simulink model "stewart_platform_model"  (R2025b)
settings: Solver=ode45  StartTime=0.0  StopTime=0.1  FixedStep=1e-4  MaxStep=0.2  RelTol=1e-4  AbsTol=1e-4
values from neighbouring files (symbols this model uses):
  ground = initializeGround('type', 'none')    [active_damping_dvf.m]    (also in active_damping_iff.m; active_damping_inertial.m; cubic_conf_coupling_cartesianl.m; cubic_conf_coupling_strutsl.m)
  payload = initializePayload('type', 'none')    [active_damping_dvf.m]    (also in active_damping_iff.m; active_damping_inertial.m; cubic_conf_coupling_cartesianl.m; cubic_conf_coupling_strutsl.m)
  s = zpk('s')    [active_damping_dvf.m]    (also in active_damping_iff.m; active_damping_inertial.m; cubic_conf_above_platforml.m; cubic_conf_coupling_cartesianl.m)
undefined symbols (not defined in the file or in its folder): X, Y, Z
libraries: sm_lib x29, nesl_utility x27, cstblocks x10
(part 2 of 2)

== system stewart_platform_model/Payload/Cartesian ==
  Cartesian Joint : sm_lib/Joints/Cartesian Joint  JointMode=Normal  CompositeWrenchDir=FollowerOnBase  CompositeWrenchFrame=BaseFrame  SenseConstraintForce=off  SenseConstraintTorque=off  SenseTotalForce=off  SenseTotalTorque=off  PxPositionTargetSpecify=off  PxPositionTargetPriority=High  PxPositionTargetValue=0  PxPositionTargetValueUnits=m  PxVelocityTargetSpecify=off  PxVelocityTargetPriority=High  PxVelocityTargetValue=0  PxVelocityTargetValueUnits=m/s  PxEquilibriumPosition=0  PxEquilibriumPositionUnits=m  PxSpringStiffness=payload.K(1)  PxSpringStiffnessUnits=N/m  PxDampingCoefficient=payload.C(1)  PxDampingCoefficientUnits=N/(m/s)  PxLowerLimitSpecify=off  PxLowerLimitBound=-1  PxLowerLimitBoundUnits=m  PxLowerLimitStiffness=1e6  PxLowerLimitStiffnessUnits=N/m  PxLowerLimitDamping=1e3  PxLowerLimitDampingUnits=N/(m/s)  PxLowerLimitTransitionRegionWidth=1e-4  PxLowerLimitTransitionRegionWidthUnits=m  PxUpperLimitSpecify=off  PxUpperLimitBound=1  PxUpperLimitBoundUnits=m  PxUpperLimitStiffness=1e6  PxUpperLimitStiffnessUnits=N/m  PxUpperLimitDamping=1e3  PxUpperLimitDampingUnits=N/(m/s)  PxUpperLimitTransitionRegionWidth=1e-4  PxUpperLimitTransitionRegionWidthUnits=m  PxTorqueActuationMode=NoTorque  PxMotionActuationMode=ComputedMotion  PxSensePosition=off  PxSenseVelocity=off  PxSenseAcceleration=off  PxSenseTorqueForce=off  PxSenseLowerLimitTorqueForce=off  PxSenseUpperLimitTorqueForce=off  PyPositionTargetSpecify=off  PyPositionTargetPriority=High  PyPositionTargetValue=0  PyPositionTargetValueUnits=m  PyVelocityTargetSpecify=off  PyVelocityTargetPriority=High  PyVelocityTargetValue=0  PyVelocityTargetValueUnits=m/s  PyEquilibriumPosition=0  PyEquilibriumPositionUnits=m  PySpringStiffness=payload.K(2)  PySpringStiffnessUnits=N/m  PyDampingCoefficient=payload.C(2)  PyDampingCoefficientUnits=N/(m/s)  PyLowerLimitSpecify=off  PyLowerLimitBound=-1  PyLowerLimitBoundUnits=m  PyLowerLimitStiffness=1e6  PyLowerLimitStiffnessUnits=N/m  PyLowerLimitDamping=1e3  PyLowerLimitDampingUnits=N/(m/s)  PyLowerLimitTransitionRegionWidth=1e-4  PyLowerLimitTransitionRegionWidthUnits=m  PyUpperLimitSpecify=off  PyUpperLimitBound=1  PyUpperLimitBoundUnits=m  PyUpperLimitStiffness=1e6  PyUpperLimitStiffnessUnits=N/m  PyUpperLimitDamping=1e3  PyUpperLimitDampingUnits=N/(m/s)  PyUpperLimitTransitionRegionWidth=1e-4  PyUpperLimitTransitionRegionWidthUnits=m  PyTorqueActuationMode=NoTorque  PyMotionActuationMode=ComputedMotion  PySensePosition=off  PySenseVelocity=off  PySenseAcceleration=off  PySenseTorqueForce=off  PySenseLowerLimitTorqueForce=off  PySenseUpperLimitTorqueForce=off  PzPositionTargetSpecify=off  PzPositionTargetPriority=High  PzPositionTargetValue=0  PzPositionTargetValueUnits=m  PzVelocityTargetSpecify=off  PzVelocityTargetPriority=High  PzVelocityTargetValue=0  PzVelocityTargetValueUnits=m/s  PzEquilibriumPosition=0  PzEquilibriumPositionUnits=m  PzSpringStiffness=payload.K(3)  PzSpringStiffnessUnits=N/m  PzDampingCoefficient=payload.C(3)  PzDampingCoefficientUnits=N/(m/s)  PzLowerLimitSpecify=off  PzLowerLimitBound=-1  PzLowerLimitBoundUnits=m  PzLowerLimitStiffness=1e6  PzLowerLimitStiffnessUnits=N/m  PzLowerLimitDamping=1e3  PzLowerLimitDampingUnits=N/(m/s)  PzLowerLimitTransitionRegionWidth=1e-4  PzLowerLimitTransitionRegionWidthUnits=m  PzUpperLimitSpecify=off  PzUpperLimitBound=1  PzUpperLimitBoundUnits=m  PzUpperLimitStiffness=1e6  PzUpperLimitStiffnessUnits=N/m  PzUpperLimitDamping=1e3  PzUpperLimitDampingUnits=N/(m/s)  PzUpperLimitTransitionRegionWidth=1e-4  PzUpperLimitTransitionRegionWidthUnits=m  PzTorqueActuationMode=NoTorque  PzMotionActuationMode=ComputedMotion  PzSensePosition=off  PzSenseVelocity=off  PzSenseAcceleration=off  PzSenseTorqueForce=off  PzSenseLowerLimitTorqueForce=off  PzSenseUpperLimitTorqueForce=off
  Cylindrical Solid : sm_lib/Body Elements/Cylindrical Solid  CylinderRadius=0.1  CylinderRadiusUnits=m  CylinderLength=2*payload.h  CylinderLengthUnits=m  ExportEntireGeometry=off  InertiaType=Custom  BasedOnType=Mass  Density=1000  DensityUnits=kg/m^3  Mass=payload.m  MassUnits=kg  CenterOfMass=[0 0 payload.h]  CenterOfMassUnits=m  MomentsOfInertia=diag(payload.I)  MomentsOfInertiaUnits=kg*m^2  ProductsOfInertia=[payload.I(2,3) payload.I(1,3) payload.I(1,2)]  ProductsOfInertiaUnits=kg*m^2  GraphicType=FromGeometry  MarkerShape=Sphere  MarkerSize=10  GraphicVisPropType=SimpleVisualProperties  GraphicDiffuseColor=[0.5 0.5 0.5]  GraphicOpacity=1.0  GraphicSpecularColor=[0.5 0.5 0.5 1.0]  GraphicAmbientColor=[0.15 0.15 0.15 1.0]  GraphicEmissiveColor=[0.0 0.0 0.0 1.0]  GraphicShininess=75  DoExposeReferenceFrame=on  SerializedFrames=<Frames/>
  Rigid Transform : sm_lib/Frames and Transforms/Rigid Transform  RotationMethod=None  FollAlignAxisA=+X  BaseAlignAxisA=+Y  FollAlignAxisB=+Y  BaseAlignAxisB=+Z  RotationStandardAxis=+Z  RotationAngle=0.0  RotationAngleUnits=deg  RotationArbitraryAxis=[0 0 1]  RotationSequenceAxes=FollowerAxes  RotationSequence=XYX  RotationSequenceAngles=[0 0 0]  RotationSequenceAnglesUnits=deg  RotationMatrix=[1 0 0; 0 1 0; 0 0 1]  Quaternion=[1 0 0 0]  TranslationMethod=StandardAxis  TranslationCartesianOffset=[0 0 0]  TranslationCartesianOffsetUnits=m  TranslationStandardAxis=+Z  TranslationStandardOffset=payload.h  TranslationStandardOffsetUnits=m  TranslationROffset=0  TranslationROffsetUnits=m  TranslationThetaOffset=0  TranslationThetaOffsetUnits=deg  TranslationZOffset=0  TranslationZOffsetUnits=m
  Rigid Transform1 : sm_lib/Frames and Transforms/Rigid Transform  RotationMethod=None  FollAlignAxisA=+X  BaseAlignAxisA=+Y  FollAlignAxisB=+Y  BaseAlignAxisB=+Z  RotationStandardAxis=+Z  RotationAngle=0.0  RotationAngleUnits=deg  RotationArbitraryAxis=[0 0 1]  RotationSequenceAxes=FollowerAxes  RotationSequence=XYX  RotationSequenceAngles=[0 0 0]  RotationSequenceAnglesUnits=deg  RotationMatrix=[1 0 0; 0 1 0; 0 0 1]  Quaternion=[1 0 0 0]  TranslationMethod=StandardAxis  TranslationCartesianOffset=[0 0 0]  TranslationCartesianOffsetUnits=m  TranslationStandardAxis=+Z  TranslationStandardOffset=payload.h  TranslationStandardOffsetUnits=m  TranslationROffset=0  TranslationROffsetUnits=m  TranslationThetaOffset=0  TranslationThetaOffsetUnits=deg  TranslationZOffset=0  TranslationZOffsetUnits=m
  Rigid Transform2 : sm_lib/Frames and Transforms/Rigid Transform  RotationMethod=None  FollAlignAxisA=+X  BaseAlignAxisA=+Y  FollAlignAxisB=+Y  BaseAlignAxisB=+Z  RotationStandardAxis=+Z  RotationAngle=0.0  RotationAngleUnits=deg  RotationArbitraryAxis=[0 0 1]  RotationSequenceAxes=FollowerAxes  RotationSequence=XYX  RotationSequenceAngles=[0 0 0]  RotationSequenceAnglesUnits=deg  RotationMatrix=[1 0 0; 0 1 0; 0 0 1]  Quaternion=[1 0 0 0]  TranslationMethod=Cartesian  TranslationCartesianOffset=stewart.platform_M.MO_B  TranslationCartesianOffsetUnits=m  TranslationStandardAxis=+Z  TranslationStandardOffset=0  TranslationStandardOffsetUnits=m  TranslationROffset=0  TranslationROffsetUnits=m  TranslationThetaOffset=0  TranslationThetaOffsetUnits=deg  TranslationZOffset=0  TranslationZOffsetUnits=m
  "{M}" : PMIOPort  Side=Left
  "{P}" : PMIOPort  Port=2  Side=Right
  connections:
  Cartesian Joint/LConn1 -- Rigid Transform/RConn1
  Rigid Transform/LConn1 -- "{M}"/RConn1
  Cartesian Joint/RConn1 -- Rigid Transform1/RConn1 -- Cylindrical Solid/RConn1
  "{P}"/RConn1 -- Rigid Transform2/RConn1
  Rigid Transform2/LConn1 -- Rigid Transform1/LConn1

== system stewart_platform_model/Payload/Flexible ==
  Bushing Joint : sm_lib/Joints/Bushing Joint  JointMode=Normal  CompositeWrenchDir=FollowerOnBase  CompositeWrenchFrame=BaseFrame  SenseConstraintForce=off  SenseConstraintTorque=off  SenseTotalForce=off  SenseTotalTorque=off  PxPositionTargetSpecify=off  PxPositionTargetPriority=High  PxPositionTargetValue=0  PxPositionTargetValueUnits=m  PxVelocityTargetSpecify=off  PxVelocityTargetPriority=High  PxVelocityTargetValue=0  PxVelocityTargetValueUnits=m/s  PxEquilibriumPosition=0  PxEquilibriumPositionUnits=m  PxSpringStiffness=payload.K(1)  PxSpringStiffnessUnits=N/m  PxDampingCoefficient=payload.C(1)  PxDampingCoefficientUnits=N/(m/s)  PxLowerLimitSpecify=off  PxLowerLimitBound=-1  PxLowerLimitBoundUnits=m  PxLowerLimitStiffness=1e6  PxLowerLimitStiffnessUnits=N/m  PxLowerLimitDamping=1e3  PxLowerLimitDampingUnits=N/(m/s)  PxLowerLimitTransitionRegionWidth=1e-4  PxLowerLimitTransitionRegionWidthUnits=m  PxUpperLimitSpecify=off  PxUpperLimitBound=1  PxUpperLimitBoundUnits=m  PxUpperLimitStiffness=1e6  PxUpperLimitStiffnessUnits=N/m  PxUpperLimitDamping=1e3  PxUpperLimitDampingUnits=N/(m/s)  PxUpperLimitTransitionRegionWidth=1e-4  PxUpperLimitTransitionRegionWidthUnits=m  PxTorqueActuationMode=NoTorque  PxMotionActuationMode=ComputedMotion  PxSensePosition=off  PxSenseVelocity=off  PxSenseAcceleration=off  PxSenseTorqueForce=off  PxSenseLowerLimitTorqueForce=off  PxSenseUpperLimitTorqueForce=off  PyPositionTargetSpecify=off  PyPositionTargetPriority=High  PyPositionTargetValue=0  PyPositionTargetValueUnits=m  PyVelocityTargetSpecify=off  PyVelocityTargetPriority=High  PyVelocityTargetValue=0  PyVelocityTargetValueUnits=m/s  PyEquilibriumPosition=0  PyEquilibriumPositionUnits=m  PySpringStiffness=payload.K(2)  PySpringStiffnessUnits=N/m  PyDampingCoefficient=payload.C(2)  PyDampingCoefficientUnits=N/(m/s)  PyLowerLimitSpecify=off  PyLowerLimitBound=-1  PyLowerLimitBoundUnits=m  PyLowerLimitStiffness=1e6  PyLowerLimitStiffnessUnits=N/m  PyLowerLimitDamping=1e3  PyLowerLimitDampingUnits=N/(m/s)  PyLowerLimitTransitionRegionWidth=1e-4  PyLowerLimitTransitionRegionWidthUnits=m  PyUpperLimitSpecify=off  PyUpperLimitBound=1  PyUpperLimitBoundUnits=m  PyUpperLimitStiffness=1e6  PyUpperLimitStiffnessUnits=N/m  PyUpperLimitDamping=1e3  PyUpperLimitDampingUnits=N/(m/s)  PyUpperLimitTransitionRegionWidth=1e-4  PyUpperLimitTransitionRegionWidthUnits=m  PyTorqueActuationMode=NoTorque  PyMotionActuationMode=ComputedMotion  PySensePosition=off  PySenseVelocity=off  PySenseAcceleration=off  PySenseTorqueForce=off  PySenseLowerLimitTorqueForce=off  PySenseUpperLimitTorqueForce=off  PzPositionTargetSpecify=off  PzPositionTargetPriority=High  PzPositionTargetValue=0  PzPositionTargetValueUnits=m  PzVelocityTargetSpecify=off  PzVelocityTargetPriority=High  PzVelocityTargetValue=0  PzVelocityTargetValueUnits=m/s  PzEquilibriumPosition=0  PzEquilibriumPositionUnits=m  PzSpringStiffness=payload.K(3)  PzSpringStiffnessUnits=N/m  PzDampingCoefficient=payload.C(3)  PzDampingCoefficientUnits=N/(m/s)  PzLowerLimitSpecify=off  PzLowerLimitBound=-1  PzLowerLimitBoundUnits=m  PzLowerLimitStiffness=1e6  PzLowerLimitStiffnessUnits=N/m  PzLowerLimitDamping=1e3  PzLowerLimitDampingUnits=N/(m/s)  PzLowerLimitTransitionRegionWidth=1e-4  PzLowerLimitTransitionRegionWidthUnits=m  PzUpperLimitSpecify=off  PzUpperLimitBound=1  PzUpperLimitBoundUnits=m  PzUpperLimitStiffness=1e6  PzUpperLimitStiffnessUnits=N/m  PzUpperLimitDamping=1e3  PzUpperLimitDampingUnits=N/(m/s)  PzUpperLimitTransitionRegionWidth=1e-4  PzUpperLimitTransitionRegionWidthUnits=m  PzTorqueActuationMode=NoTorque  PzMotionActuationMode=ComputedMotion  PzSensePosition=off  PzSenseVelocity=off  PzSenseAcceleration=off  PzSenseTorqueForce=off  PzSenseLowerLimitTorqueForce=off  PzSenseUpperLimitTorqueForce=off  RxPositionTargetSpecify=off  RxPositionTargetPriority=High  RxPositionTargetValue=0  RxPositionTargetValueUnits=deg  RxVelocityTargetSpecify=off  RxVelocityTargetPriority=High  RxVelocityTargetValue=0  RxVelocityTargetValueUnits=deg/s  RxEquilibriumPosition=0  RxEquilibriumPositionUnits=deg  RxSpringStiffness=payload.K(4)  RxSpringStiffnessUnits=N*m/rad  RxDampingCoefficient=payload.C(4)  RxDampingCoefficientUnits=N*m/(rad/s)  RxLowerLimitSpecify=off  RxLowerLimitBound=-90  RxLowerLimitBoundUnits=deg  RxLowerLimitStiffness=1e4  RxLowerLimitStiffnessUnits=N*m/deg  RxLowerLimitDamping=10  RxLowerLimitDampingUnits=N*m/(deg/s)  RxLowerLimitTransitionRegionWidth=0.1  RxLowerLimitTransitionRegionWidthUnits=deg  RxUpperLimitSpecify=off  RxUpperLimitBound=90  RxUpperLimitBoundUnits=deg  RxUpperLimitStiffness=1e4  RxUpperLimitStiffnessUnits=N*m/deg  RxUpperLimitDamping=10  RxUpperLimitDampingUnits=N*m/(deg/s)  RxUpperLimitTransitionRegionWidth=0.1  RxUpperLimitTransitionRegionWidthUnits=deg  RxTorqueActuationMode=NoTorque  RxMotionActuationMode=ComputedMotion  RxSensePosition=off  RxSenseVelocity=off  RxSenseAcceleration=off  RxSenseTorqueForce=off  RxSenseLowerLimitTorqueForce=off  RxSenseUpperLimitTorqueForce=off  RyPositionTargetSpecify=off  RyPositionTargetPriority=High  RyPositionTargetValue=0  RyPositionTargetValueUnits=deg  RyVelocityTargetSpecify=off  RyVelocityTargetPriority=High  RyVelocityTargetValue=0  RyVelocityTargetValueUnits=deg/s  RyEquilibriumPosition=0  RyEquilibriumPositionUnits=deg  RySpringStiffness=payload.K(5)  RySpringStiffnessUnits=N*m/rad  RyDampingCoefficient=payload.C(5)  RyDampingCoefficientUnits=N*m/(rad/s)  RyLowerLimitSpecify=off  RyLowerLimitBound=-90  RyLowerLimitBoundUnits=deg  RyLowerLimitStiffness=1e4  RyLowerLimitStiffnessUnits=N*m/deg  RyLowerLimitDamping=10  RyLowerLimitDampingUnits=N*m/(deg/s)  RyLowerLimitTransitionRegionWidth=0.1  RyLowerLimitTransitionRegionWidthUnits=deg  RyUpperLimitSpecify=off  RyUpperLimitBound=90  RyUpperLimitBoundUnits=deg  RyUpperLimitStiffness=1e4  RyUpperLimitStiffnessUnits=N*m/deg  RyUpperLimitDamping=10  RyUpperLimitDampingUnits=N*m/(deg/s)  RyUpperLimitTransitionRegionWidth=0.1  RyUpperLimitTransitionRegionWidthUnits=deg  RyTorqueActuationMode=NoTorque  RyMotionActuationMode=ComputedMotion  RySensePosition=off  RySenseVelocity=off  RySenseAcceleration=off  RySenseTorqueForce=off  RySenseLowerLimitTorqueForce=off  RySenseUpperLimitTorqueForce=off  RzPositionTargetSpecify=off  RzPositionTargetPriority=High  RzPositionTargetValue=0  RzPositionTargetValueUnits=deg  RzVelocityTargetSpecify=off  RzVelocityTargetPriority=High  RzVelocityTargetValue=0  RzVelocityTargetValueUnits=deg/s  RzEquilibriumPosition=0  RzEquilibriumPositionUnits=deg  RzSpringStiffness=payload.K(6)  RzSpringStiffnessUnits=N*m/rad  RzDampingCoefficient=payload.C(6)  RzDampingCoefficientUnits=N*m/(rad/s)  RzLowerLimitSpecify=off  RzLowerLimitBound=-90  RzLowerLimitBoundUnits=deg  RzLowerLimitStiffness=1e4  RzLowerLimitStiffnessUnits=N*m/deg  RzLowerLimitDamping=10  RzLowerLimitDampingUnits=N*m/(deg/s)  RzLowerLimitTransitionRegionWidth=0.1  RzLowerLimitTransitionRegionWidthUnits=deg  RzUpperLimitSpecify=off  RzUpperLimitBound=90  RzUpperLimitBoundUnits=deg  RzUpperLimitStiffness=1e4  RzUpperLimitStiffnessUnits=N*m/deg  RzUpperLimitDamping=10  RzUpperLimitDampingUnits=N*m/(deg/s)  RzUpperLimitTransitionRegionWidth=0.1  RzUpperLimitTransitionRegionWidthUnits=deg  RzTorqueActuationMode=NoTorque  RzMotionActuationMode=ComputedMotion  RzSensePosition=off  RzSenseVelocity=off  RzSenseAcceleration=off  RzSenseTorqueForce=off  RzSenseLowerLimitTorqueForce=off  RzSenseUpperLimitTorqueForce=off
  Cylindrical Solid : sm_lib/Body Elements/Cylindrical Solid  CylinderRadius=0.1  CylinderRadiusUnits=m  CylinderLength=2*payload.h  CylinderLengthUnits=m  ExportEntireGeometry=off  InertiaType=Custom  BasedOnType=Mass  Density=1000  DensityUnits=kg/m^3  Mass=payload.m  MassUnits=kg  CenterOfMass=[0 0 payload.h]  CenterOfMassUnits=m  MomentsOfInertia=diag(payload.I)  MomentsOfInertiaUnits=kg*m^2  ProductsOfInertia=[payload.I(2,3) payload.I(1,3) payload.I(1,2)]  ProductsOfInertiaUnits=kg*m^2  GraphicType=FromGeometry  MarkerShape=Sphere  MarkerSize=10  GraphicVisPropType=SimpleVisualProperties  GraphicDiffuseColor=[0.5 0.5 0.5]  GraphicOpacity=1.0  GraphicSpecularColor=[0.5 0.5 0.5 1.0]  GraphicAmbientColor=[0.15 0.15 0.15 1.0]  GraphicEmissiveColor=[0.0 0.0 0.0 1.0]  GraphicShininess=75  DoExposeReferenceFrame=on  SerializedFrames=<Frames/>
  Rigid Transform : sm_lib/Frames and Transforms/Rigid Transform  RotationMethod=None  FollAlignAxisA=+X  BaseAlignAxisA=+Y  FollAlignAxisB=+Y  BaseAlignAxisB=+Z  RotationStandardAxis=+Z  RotationAngle=0.0  RotationAngleUnits=deg  RotationArbitraryAxis=[0 0 1]  RotationSequenceAxes=FollowerAxes  RotationSequence=XYX  RotationSequenceAngles=[0 0 0]  RotationSequenceAnglesUnits=deg  RotationMatrix=[1 0 0; 0 1 0; 0 0 1]  Quaternion=[1 0 0 0]  TranslationMethod=StandardAxis  TranslationCartesianOffset=[0 0 0]  TranslationCartesianOffsetUnits=m  TranslationStandardAxis=+Z  TranslationStandardOffset=payload.h  TranslationStandardOffsetUnits=m  TranslationROffset=0  TranslationROffsetUnits=m  TranslationThetaOffset=0  TranslationThetaOffsetUnits=deg  TranslationZOffset=0  TranslationZOffsetUnits=m
  Rigid Transform1 : sm_lib/Frames and Transforms/Rigid Transform  RotationMethod=None  FollAlignAxisA=+X  BaseAlignAxisA=+Y  FollAlignAxisB=+Y  BaseAlignAxisB=+Z  RotationStandardAxis=+Z  RotationAngle=0.0  RotationAngleUnits=deg  RotationArbitraryAxis=[0 0 1]  RotationSequenceAxes=FollowerAxes  RotationSequence=XYX  RotationSequenceAngles=[0 0 0]  RotationSequenceAnglesUnits=deg  RotationMatrix=[1 0 0; 0 1 0; 0 0 1]  Quaternion=[1 0 0 0]  TranslationMethod=StandardAxis  TranslationCartesianOffset=[0 0 0]  TranslationCartesianOffsetUnits=m  TranslationStandardAxis=+Z  TranslationStandardOffset=payload.h  TranslationStandardOffsetUnits=m  TranslationROffset=0  TranslationROffsetUnits=m  TranslationThetaOffset=0  TranslationThetaOffsetUnits=deg  TranslationZOffset=0  TranslationZOffsetUnits=m
  Rigid Transform2 : sm_lib/Frames and Transforms/Rigid Transform  RotationMethod=None  FollAlignAxisA=+X  BaseAlignAxisA=+Y  FollAlignAxisB=+Y  BaseAlignAxisB=+Z  RotationStandardAxis=+Z  RotationAngle=0.0  RotationAngleUnits=deg  RotationArbitraryAxis=[0 0 1]  RotationSequenceAxes=FollowerAxes  RotationSequence=XYX  RotationSequenceAngles=[0 0 0]  RotationSequenceAnglesUnits=deg  RotationMatrix=[1 0 0; 0 1 0; 0 0 1]  Quaternion=[1 0 0 0]  TranslationMethod=Cartesian  TranslationCartesianOffset=stewart.platform_M.MO_B  TranslationCartesianOffsetUnits=m  TranslationStandardAxis=+Z  TranslationStandardOffset=0  TranslationStandardOffsetUnits=m  TranslationROffset=0  TranslationROffsetUnits=m  TranslationThetaOffset=0  TranslationThetaOffsetUnits=deg  TranslationZOffset=0  TranslationZOffsetUnits=m
  "{M}" : PMIOPort  Side=Left
  "{P}" : PMIOPort  Port=2  Side=Right
  connections:
  Cylindrical Solid/RConn1 -- Rigid Transform1/RConn1 -- Bushing Joint/RConn1
  Rigid Transform/LConn1 -- "{M}"/RConn1
  Bushing Joint/LConn1 -- Rigid Transform/RConn1
  Rigid Transform2/LConn1 -- Rigid Transform1/LConn1
  "{P}"/RConn1 -- Rigid Transform2/RConn1

== system stewart_platform_model/Payload/None ==
  Rigid Transform2 : sm_lib/Frames and Transforms/Rigid Transform  RotationMethod=None  FollAlignAxisA=+X  BaseAlignAxisA=+Y  FollAlignAxisB=+Y  BaseAlignAxisB=+Z  RotationStandardAxis=+Z  RotationAngle=0.0  RotationAngleUnits=deg  RotationArbitraryAxis=[0 0 1]  RotationSequenceAxes=FollowerAxes  RotationSequence=XYX  RotationSequenceAngles=[0 0 0]  RotationSequenceAnglesUnits=deg  RotationMatrix=[1 0 0; 0 1 0; 0 0 1]  Quaternion=[1 0 0 0]  TranslationMethod=Cartesian  TranslationCartesianOffset=stewart.platform_M.MO_B  TranslationCartesianOffsetUnits=m  TranslationStandardAxis=+Z  TranslationStandardOffset=0  TranslationStandardOffsetUnits=m  TranslationROffset=0  TranslationROffsetUnits=m  TranslationThetaOffset=0  TranslationThetaOffsetUnits=deg  TranslationZOffset=0  TranslationZOffsetUnits=m
  "{M}" : PMIOPort  Side=Left
  "{P}" : PMIOPort  Port=2  Side=Right
  connections:
  "{P}"/RConn1 -- Rigid Transform2/RConn1
  Rigid Transform2/LConn1 -- "{M}"/RConn1

== system stewart_platform_model/Payload/Rigid ==
  Cylindrical Solid : sm_lib/Body Elements/Cylindrical Solid  CylinderRadius=0.1  CylinderRadiusUnits=m  CylinderLength=2*payload.h  CylinderLengthUnits=m  ExportEntireGeometry=off  InertiaType=Custom  BasedOnType=Mass  Density=1000  DensityUnits=kg/m^3  Mass=payload.m  MassUnits=kg  CenterOfMass=[0 0 payload.h]  CenterOfMassUnits=m  MomentsOfInertia=diag(payload.I)  MomentsOfInertiaUnits=kg*m^2  ProductsOfInertia=[payload.I(2,3) payload.I(1,3) payload.I(1,2)]  ProductsOfInertiaUnits=kg*m^2  GraphicType=FromGeometry  MarkerShape=Sphere  MarkerSize=10  GraphicVisPropType=SimpleVisualProperties  GraphicDiffuseColor=[0.5019608 0.85882354 0.6901961]  GraphicOpacity=1.0  GraphicSpecularColor=[0.5 0.5 0.5 1.0]  GraphicAmbientColor=[0.15 0.15 0.15 1.0]  GraphicEmissiveColor=[0.0 0.0 0.0 1.0]  GraphicShininess=75  DoExposeReferenceFrame=on  SerializedFrames=<Frames/>
  Rigid Transform : sm_lib/Frames and Transforms/Rigid Transform  RotationMethod=None  FollAlignAxisA=+X  BaseAlignAxisA=+Y  FollAlignAxisB=+Y  BaseAlignAxisB=+Z  RotationStandardAxis=+Z  RotationAngle=0.0  RotationAngleUnits=deg  RotationArbitraryAxis=[0 0 1]  RotationSequenceAxes=FollowerAxes  RotationSequence=XYX  RotationSequenceAngles=[0 0 0]  RotationSequenceAnglesUnits=deg  RotationMatrix=[1 0 0; 0 1 0; 0 0 1]  Quaternion=[1 0 0 0]  TranslationMethod=StandardAxis  TranslationCartesianOffset=[0 0 0]  TranslationCartesianOffsetUnits=m  TranslationStandardAxis=+Z  TranslationStandardOffset=payload.h  TranslationStandardOffsetUnits=m  TranslationROffset=0  TranslationROffsetUnits=m  TranslationThetaOffset=0  TranslationThetaOffsetUnits=deg  TranslationZOffset=0  TranslationZOffsetUnits=m
  Rigid Transform2 : sm_lib/Frames and Transforms/Rigid Transform  RotationMethod=None  FollAlignAxisA=+X  BaseAlignAxisA=+Y  FollAlignAxisB=+Y  BaseAlignAxisB=+Z  RotationStandardAxis=+Z  RotationAngle=0.0  RotationAngleUnits=deg  RotationArbitraryAxis=[0 0 1]  RotationSequenceAxes=FollowerAxes  RotationSequence=XYX  RotationSequenceAngles=[0 0 0]  RotationSequenceAnglesUnits=deg  RotationMatrix=[1 0 0; 0 1 0; 0 0 1]  Quaternion=[1 0 0 0]  TranslationMethod=Cartesian  TranslationCartesianOffset=stewart.platform_M.MO_B  TranslationCartesianOffsetUnits=m  TranslationStandardAxis=+Z  TranslationStandardOffset=0  TranslationStandardOffsetUnits=m  TranslationROffset=0  TranslationROffsetUnits=m  TranslationThetaOffset=0  TranslationThetaOffsetUnits=deg  TranslationZOffset=0  TranslationZOffsetUnits=m
  "{M}" : PMIOPort  Side=Left
  "{P}" : PMIOPort  Port=2  Side=Right
  connections:
  Rigid Transform/LConn1 -- Rigid Transform2/LConn1 -- "{M}"/RConn1
  Cylindrical Solid/RConn1 -- Rigid Transform/RConn1
  "{P}"/RConn1 -- Rigid Transform2/RConn1

== matlab function stewart_platform_model/Absolute Motion Sensor/MATLAB Function ==
  data: rotm input; Rx output; Ry output; Rz output
function [Rx, Ry, Rz] = fcn(rotm)

    if (rotm(3,1) < 1)
        if (rotm(3,1) > -1) % case 1: if r31 ~= ±1
            % Solution with positive sign. It limits the range of the values
            % of theta_y to (-pi/2, pi/2):
            Rz = atan2(rotm(2,1), rotm(1,1)); % theta_z
            Ry = asin(-rotm(3,1));            % theta_y
            Rx = atan2(rotm(3,2), rotm(3,3)); % theta_x
        else % case 2: if r31 = -1
            % theta_x and theta_z are linked --> Gimbal lock:
            % There are infinity number of solutions for theta_x - theta_z = atan2(-r23, r22).
            % To find a solution, set theta_x = 0 by convention.
            Rz = -atan2(-rotm(2,3), rotm(2,2));
            Ry = pi/2;
            Rx = 0;
        end
    else % case 3: if r31 = 1
        % Gimbal lock: There is not a unique solution for
        %   theta_x + theta_z = atan2(-r23, r22), by convention, set theta_x = 0.
        Rz = atan2(-rotm(2,3), rotm(2,2));
        Ry = -pi/2;
        Rx = 0;
    end

== matlab function stewart_platform_model/Relative Motion Sensor/MATLAB Function ==
  data: rotm input; Rx output; Ry output; Rz output
function [Rx, Ry, Rz] = fcn(rotm)

    if (rotm(3,1) < 1)
        if (rotm(3,1) > -1) % case 1: if r31 ~= ±1
            % Solution with positive sign. It limits the range of the values
            % of theta_y to (-pi/2, pi/2):
            Rz = atan2(rotm(2,1), rotm(1,1)); % theta_z
            Ry = asin(-rotm(3,1));            % theta_y
            Rx = atan2(rotm(3,2), rotm(3,3)); % theta_x
        else % case 2: if r31 = -1
            % theta_x and theta_z are linked --> Gimbal lock:
            % There are infinity number of solutions for theta_x - theta_z = atan2(-r23, r22).
            % To find a solution, set theta_x = 0 by convention.
            Rz = -atan2(-rotm(2,3), rotm(2,2));
            Ry = pi/2;
            Rx = 0;
        end
    else % case 3: if r31 = 1
        % Gimbal lock: There is not a unique solution for
        %   theta_x + theta_z = atan2(-r23, r22), by convention, set theta_x = 0.
        Rz = atan2(-rotm(2,3), rotm(2,2));
        Ry = -pi/2;
        Rx = 0;
    end

== matlab function stewart_platform_model/Controller/Reference-Tracking-X/MATLAB Function3 ==
  data: Dxr input; Edx output; Dyr input; Dzr input; Rxr input; Ryr input; Rzr input; Dxm input; Dym input; Dzm input; Rxm input; Rym input; Rzm input; Edy output; Edz output; Erx output; Ery output; Erz output
function [Edx, Edy, Edz, Erx, Ery, Erz] = computePositionError(Dxr, Dyr, Dzr, Rxr, Ryr, Rzr, Dxm, Dym, Dzm, Rxm, Rym, Rzm)

%% Measured Pose
WTm = zeros(4,4);

WTm(1:3, 1:3) = [cos(Rzm) -sin(Rzm) 0;
     sin(Rzm)  cos(Rzm) 0;
     0        0         1] * ...
    [cos(Rym)  0        sin(Rym);
     0        1        0;
     -sin(Rym)  0        cos(Rym)] * ...
    [1        0        0;
     0        cos(Rxm) -sin(Rxm);
     0        sin(Rxm)  cos(Rxm)];
WTm(1:4, 4) = [Dxm ; Dym ; Dzm; 1];

%% Reference Pose
WTr = zeros(4,4);

WTr(1:3, 1:3) = [cos(Rzr) -sin(Rzr) 0;
     sin(Rzr)  cos(Rzr) 0;
     0        0         1] * ...
    [cos(Ryr)  0        sin(Ryr);
     0        1        0;
     -sin(Ryr)  0        cos(Ryr)] * ...
    [1        0        0;
     0        cos(Rxr) -sin(Rxr);
     0        sin(Rxr)  cos(Rxr)];
WTr(1:4, 4) = [Dxr ; Dyr ; Dzr; 1];

WTv = eye(4);
WTv(1:3, 4) = WTm(1:3, 4);

%% Wanted pose expressed in a frame corresponding to the actual measured pose
MTr = [WTm(1:3,1:3)', -WTm(1:3,1:3)'*WTm(1:3,4) ; 0 0 0 1]*WTr;

%% Extract Translations and Rotations from the Homogeneous Matrix
T = MTr;
Edx = T(1, 4);
Edy = T(2, 4);
Edz = T(3, 4);

% The angles obtained are u-v-w Euler angles (rotations in the moving frame)
Ery = atan2( T(1, 3),          sqrt(T(1, 1)^2 + T(1, 2)^2));
Erx = atan2(-T(2, 3)/cos(Ery), T(3, 3)/cos(Ery));
Erz = atan2(-T(1, 2)/cos(Ery), T(1, 1)/cos(Ery));
end

== matlab function stewart_platform_model/Controller/Reference-Tracking-HAC-DVF/MATLAB Function3 ==
  data: Dxr input; Edx output; Dyr input; Dzr input; Rxr input; Ryr input; Rzr input; Dxm input; Dym input; Dzm input; Rxm input; Rym input; Rzm input; Edy output; Edz output; Erx output; Ery output; Erz output
function [Edx, Edy, Edz, Erx, Ery, Erz] = computePositionError(Dxr, Dyr, Dzr, Rxr, Ryr, Rzr, Dxm, Dym, Dzm, Rxm, Rym, Rzm)

%% Measured Pose
WTm = zeros(4,4);

WTm(1:3, 1:3) = [cos(Rzm) -sin(Rzm) 0;
     sin(Rzm)  cos(Rzm) 0;
     0        0         1] * ...
    [cos(Rym)  0        sin(Rym);
     0        1        0;
     -sin(Rym)  0        cos(Rym)] * ...
    [1        0        0;
     0        cos(Rxm) -sin(Rxm);
     0        sin(Rxm)  cos(Rxm)];
WTm(1:4, 4) = [Dxm ; Dym ; Dzm; 1];

%% Reference Pose
WTr = zeros(4,4);

WTr(1:3, 1:3) = [cos(Rzr) -sin(Rzr) 0;
     sin(Rzr)  cos(Rzr) 0;
     0        0         1] * ...
    [cos(Ryr)  0        sin(Ryr);
     0        1        0;
     -sin(Ryr)  0        cos(Ryr)] * ...
    [1        0        0;
     0        cos(Rxr) -sin(Rxr);
     0        sin(Rxr)  cos(Rxr)];
WTr(1:4, 4) = [Dxr ; Dyr ; Dzr; 1];

WTv = eye(4);
WTv(1:3, 4) = WTm(1:3, 4);

%% Wanted pose expressed in a frame corresponding to the actual measured pose
MTr = [WTm(1:3,1:3)', -WTm(1:3,1:3)'*WTm(1:3,4) ; 0 0 0 1]*WTr;

%% Extract Translations and Rotations from the Homogeneous Matrix
T = MTr;
Edx = T(1, 4);
Edy = T(2, 4);
Edz = T(3, 4);

% The angles obtained are u-v-w Euler angles (rotations in the moving frame)
Ery = atan2( T(1, 3),          sqrt(T(1, 1)^2 + T(1, 2)^2));
Erx = atan2(-T(2, 3)/cos(Ery), T(3, 3)/cos(Ery));
Erz = atan2(-T(1, 2)/cos(Ery), T(1, 1)/cos(Ery));
end
